simulink subsystem "Kinematics"  (R2024b)
settings: Solver=VariableStepAuto  StartTime=0.0  StopTime=10.0  RelTol=1e-3
settings Model: Creator=marco  LastModifiedBy=ferru

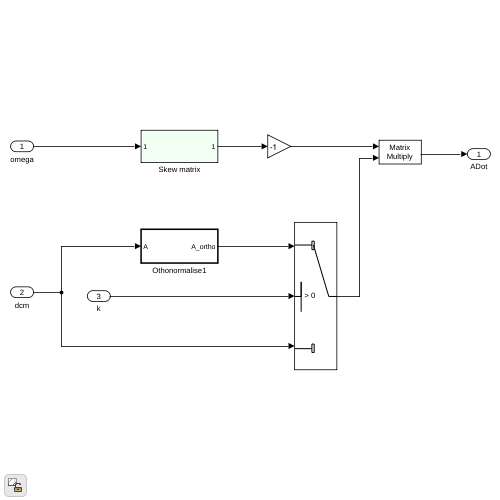
[thumbnail: Simulink's stored preview of the top-level diagram]
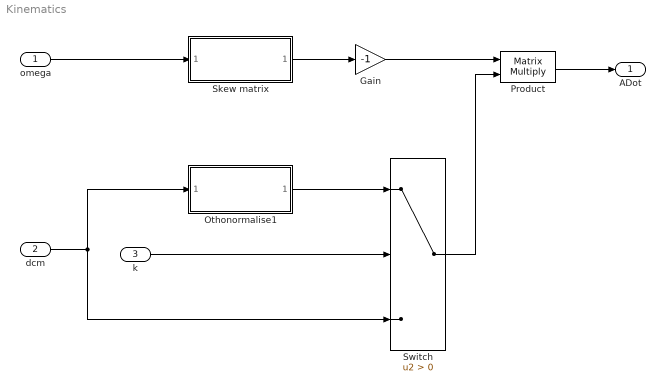
== system Kinematics ==
  omega : Inport
  dcm : Inport  Port=2
  k : Inport  Port=3
  Gain : Gain  Gain=-1
  Othonormalise1 : Subsystem  TreatAsAtomicUnit=on  ReferencedSubsystem=Othonormalise
  Product : Product  Multiplication=Matrix(*)
  Skew matrix : Subsystem  ReferencedSubsystem=SkewMatrix
  Switch : Switch  Criteria=u2 > Threshold  SaturateOnIntegerOverflow=off  InputSameDT=off
  ADot : Outport
  wires:
  Product/1 -> ADot/1
  Gain/1 -> Product/1
  Skew matrix/1 -> Gain/1
  omega/1 -> Skew matrix/1
  dcm/1 -> Switch/3, Othonormalise1/1
  k/1 -> Switch/2
  Othonormalise1/1 -> Switch/1
  Switch/1 -> Product/2
